simulink model "sf_launchabort"  (R2025b)
settings: Solver=FixedStepDiscrete  StartTime=0.0  StopTime=136  RelTol=1e-3
libraries: SignalEditorBlockLib x1
settings Model: Creator=The MathWorks, Inc.  LastModifiedBy=The MathWorks, Inc.
settings SolverCC: AlgebraicLoopSolver=TrustRegion
settings DataIOCC: LimitDataPoints=on  SaveFormat=Array  ReturnWorkspaceOutputs=off
settings OptimizationCC: ReuseModelBlockBuffer=off  ExpressionDepthLimit=2147483647.0  InitFltsAndDblsToZero=on  EfficientMapNaN2IntZero=off  LifeSpan=1  EfficientTunableParamExpr=on
settings DebuggingCC: SaveWithParameterizedLinksMsg=none  UnderspecifiedInitializationDetection=Classic  MergeDetectMultiDrivingBlocksExec=none  SignalResolutionControl=TryResolveAllWithWarning  FcnCallInpInsideContextMsg=warning  UnconnectedInputMsg=warning  UnconnectedOutputMsg=warning  UnconnectedLineMsg=warning  StateNameClashWarn=warning  SFUnexpectedBacktrackingDiag=warning  SFNoUnconditionalDefaultTransitionDiag=warning  SFExecutionAtInitializationDiag=none  ArithmeticOperatorsInVariantConditions=warning
settings HardwareCC: ProdBitPerPointer=32.0  ProdBitPerSizeT=32.0  ProdBitPerPtrDiffT=32.0  ProdLargestAtomicFloat=None  ProdIntDivRoundTo=Undefined  ProdEndianess=Unspecified  ProdWordSize=32.0  ProdHWDeviceType=32-bit Generic
settings ModelReferenceCC: EnableRefExpFcnMdlSchedulingChecks=on  PropagateSignalLabelsOutOfModel=off
settings SFSimCC: SimUseLocalCustomCode=off  SimParseCustomCode=off  CustomCodeUndefinedFunction=UseInterfaceOnly
settings RTWCC: SystemTargetFile=ert.tlc  GenCodeOnly=on  TemplateMakefile=ert_default_tmf  GenerateReport=on  RTWUseLocalCustomCode=off  IncludeHyperlinkInReport=on  LaunchReport=on  GPUComputeCapability=3.5  DLArmComputeVersion=19.05  Description=Real-Time Workshop Embedded Coder (no auto configuration)
settings CodeAppCC: IgnoreCustomStorageClasses=off  CustomSymbolStrGlobalVar=$N$M  CustomSymbolStrType=$N$M  CustomSymbolStrFcn=$N$M$F  CustomSymbolStrModelFcn=$N  CustomSymbolStrMacro=$N$M  StateflowObjectComments=on  InternalIdentifier=Classic
settings ERTTargetCC: InlinedParameterPlacement=Hierarchical  ERTCustomFileTemplate=example_file_process.tlc  ConvertIfToSwitch=off  SuppressUnreachableDefaultCases=off  DynamicArrayContainerType=coder::array  TargetFcnLib=ansi_tfl_tmw.mat  MultiwordLength=2048.0  GenerateSampleERTMain=on  SupportContinuousTime=on
settings ConfigComp: CovScope=Subsystem  CovPath=/launchAbortController  CovMetricSettings=dcmrw  CovSaveCumulativeToWorkspaceVar=on  CovSaveSingleToWorkspaceVar=on  CovExternalEMLEnable=off

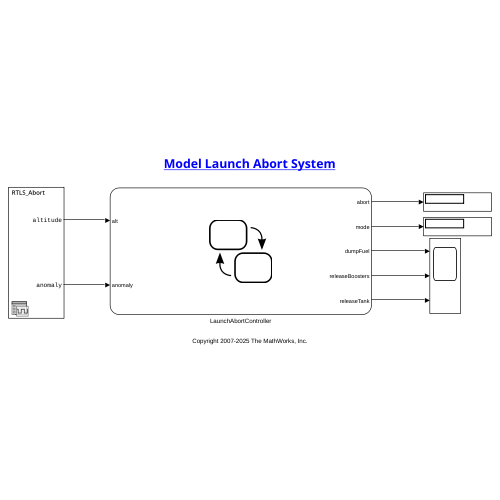
[thumbnail: Simulink's stored preview of the top-level diagram]
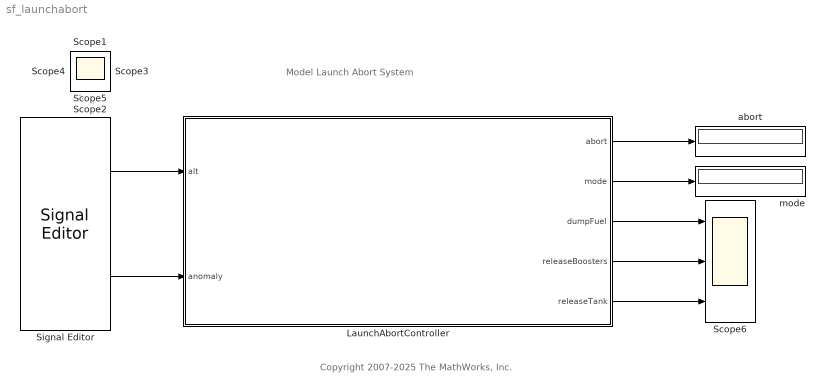
== system sf_launchabort ==
  note: Copyright 2007-2025 The MathWorks, Inc.
  note: Model Launch Abort System
  LaunchAbortController : Stateflow chart  TreatAsAtomicUnit=on
      settings: RTWSystemCode=Reusable function  RTWFcnNameOpts=Use subsystem name  RTWFileNameOpts=Use subsystem name
  Scope6 : Scope  NumInputPorts=3
      settings: ActiveDisplayYMinimum=-0.125  ActiveDisplayYMaximum=1.125
  Signal Editor : SignalEditorBlockLib/Signal Editor  FileName=LaunchAbortInput.mat  ActiveScenario=RTLS_Abort  ActiveSignal=anomaly  IsBus=off  OutputBusObjectStr=Bus: BusObject  SampleTime=0  OutputAfterFinalValue=Extrapolation  Unit=inherit  PreserveSignalName=on  ApplySigPropsToAllScenarios=on  ApplySigPropsToAllSignals=off  SignalPropertySource=Dialog parameters
  abort : Display
  mode : Display
  Scope{,1..5} (6 alike) : Scope
      Scope settings: DataLoggingMaxPoints=7500  DataLoggingSaveFormat=Array
      Scope1 settings: DataLoggingMaxPoints=7500  DataLoggingSaveFormat=Array
      Scope2 settings: ActiveDisplayYMinimum=-250  ActiveDisplayYMaximum=2750  DataLoggingMaxPoints=7500  DataLoggingVariableName=ScopeData2  DataLoggingSaveFormat=Array
      Scope3 settings: ActiveDisplayYMinimum=-250  ActiveDisplayYMaximum=2750  DataLoggingMaxPoints=7500  DataLoggingVariableName=ScopeData3  DataLoggingSaveFormat=Array
      Scope4 settings: ActiveDisplayYMinimum=-250  ActiveDisplayYMaximum=2750  DataLoggingMaxPoints=7500  DataLoggingVariableName=ScopeData4  DataLoggingSaveFormat=Array
      Scope5 settings: ActiveDisplayYMinimum=0  ActiveDisplayYMaximum=60  DataLoggingMaxPoints=7500  DataLoggingVariableName=ScopeData5  DataLoggingSaveFormat=Array
  wires:
  Signal Editor/1 -> LaunchAbortController/1(alt)
  Signal Editor/2 -> LaunchAbortController/2(anomaly)
  LaunchAbortController/2(" mode") -> mode/1
  LaunchAbortController/1(" abort") -> abort/1
  LaunchAbortController/3(dumpFuel) -> Scope6/1
  LaunchAbortController/4(releaseBoosters) -> Scope6/2
  LaunchAbortController/5(releaseTank) -> Scope6/3

== stateflow chart sf_launchabort/LaunchAbortController ==
  settings: updateMethod=DISCRETE  sampleTime=1
  state ModeLogic [parallel]
    settings: executionOrder=1
    state ReturnToLaunchSite
    state DownrangeLanding
    state AbortToOrbit
    state AbortOnceAround
    (default) -> ReturnToLaunchSite
    ReturnToLaunchSite -> DownrangeLanding : [alt>10000 && !anomaly]
    DownrangeLanding -> AbortOnceAround : [alt>100000 && !anomaly]
    AbortOnceAround -> AbortToOrbit : [alt>400000 && !anomaly]
  state Abort [parallel]
    settings: executionOrder=2
    state Normal
    state AbortLogic
      state FuelDump
        entry: dumpFuel;
      state BoosterRelease
        entry: releaseBoosters;
      state TankRelease
        entry: releaseTank;
      state NoActionRequired
      48 -> (junction 31)
      (junction 31) -> FuelDump [order 1] : [in(ModeLogic.ReturnToLaunchSite)]
      (junction 31) -> (junction 54) [order 2]
      FuelDump -> BoosterRelease : after(10,tick)
      (junction 54) -> BoosterRelease [order 1] : [in(ModeLogic.DownrangeLanding)]
      (junction 54) -> (junction 52) [order 2]
      BoosterRelease -> TankRelease : after(10,tick)
      (junction 52) -> TankRelease [order 1] : [in(ModeLogic.AbortOnceAround)]
      (junction 52) -> NoActionRequired [order 2]
      TankRelease -> (junction 32)
      NoActionRequired -> (junction 32)
      (junction 32) -> 50
    state AbortComplete
    (default) -> Normal
    Normal -> 49 : [anomaly]
    51 -> AbortComplete
  data: abort output Enum: AbortType; alt input; anomaly input; mode output Enum: ModeType
  events: dumpFuel output EITHER_EDGE_EVENT; releaseBoosters output EITHER_EDGE_EVENT; releaseTank output EITHER_EDGE_EVENT
